simulink model "SITRA_S2_test_ControllerCompare"  (R2026a)
settings: Solver=FixedStepDiscrete  StartTime=0  StopTime=600  FixedStep=1
PreLoadFcn:
  | try, mdlPath = get_param(bdroot, 'FileName'); if ~isempty(mdlPath), [pDir, ~, ~] = fileparts(mdlPath); else, pDir = pwd; end, expDir = fullfile(pDir, 'Results', 'T6_Simulink_Exports'); if ~exist(expDir, 'dir'), expDir = fullfile(pwd, 'Results', 'T6_Simulink_Exports'); end, if exist(fullfile(expDir, 'SITRA_T6.mat'), 'file'),   sref = load(fullfile(expDir, 'SITRA_T6.mat')); if isfield(sref, 'S'), sref = sref.S; end;   assignin('base', 'T6_arrivals', sref.arrivals); end, cNames = {'Webster', 'Actuated', 'MaxPressure'}; for ci = 1:numel(cNames),   cn = cNames{ci}; mf = fullfile(expDir, [cn '_T6.mat']);   if exist(mf, 'file'),     s = load(mf); if isfield(s, 'S'), s = s.S; end;     assignin('base', ['active_' cn], s.active);     assignin('base', ['gates_' cn], s.gates);   end; end, if ~evalin('base', 'exist(''SITRA_ControllerSelect'', ''var'')'), assignin('base', 'SITRA_ControllerSelect', 1); end, if ~evalin('base', 'exist(''Ceq'', ''var'')'), assignin('base', 'Ceq', 1); end, if ~evalin('base', 'exist(''kq'', ''var'')'), assignin('base', 'kq', 1); end, if ~evalin('base', 'exist(''kI'', ''var'')'), assignin('base', 'kI', 1); end, if ~evalin('base', 'exist(''traffic_dt'', ''var'')'), assignin('base', 'traffic_dt', 1); end, if ~evalin('base', 'exist(''branchCapacity'', ''var'')'), assignin('base', 'branchCapacity', [0.65; 0.35; 0.25; 0.45]); end; catch err, warning('InitFcn warning: %s', err.message); end
InitFcn:
  | try, mdlPath = get_param(bdroot, 'FileName'); if ~isempty(mdlPath), [pDir, ~, ~] = fileparts(mdlPath); else, pDir = pwd; end, expDir = fullfile(pDir, 'Results', 'T6_Simulink_Exports'); if ~exist(expDir, 'dir'), expDir = fullfile(pwd, 'Results', 'T6_Simulink_Exports'); end, if exist(fullfile(expDir, 'SITRA_T6.mat'), 'file'),   sref = load(fullfile(expDir, 'SITRA_T6.mat')); if isfield(sref, 'S'), sref = sref.S; end;   assignin('base', 'T6_arrivals', sref.arrivals); end, cNames = {'Webster', 'Actuated', 'MaxPressure'}; for ci = 1:numel(cNames),   cn = cNames{ci}; mf = fullfile(expDir, [cn '_T6.mat']);   if exist(mf, 'file'),     s = load(mf); if isfield(s, 'S'), s = s.S; end;     assignin('base', ['active_' cn], s.active);     assignin('base', ['gates_' cn], s.gates);   end; end, if ~evalin('base', 'exist(''SITRA_ControllerSelect'', ''var'')'), assignin('base', 'SITRA_ControllerSelect', 1); end, if ~evalin('base', 'exist(''Ceq'', ''var'')'), assignin('base', 'Ceq', 1); end, if ~evalin('base', 'exist(''kq'', ''var'')'), assignin('base', 'kq', 1); end, if ~evalin('base', 'exist(''kI'', ''var'')'), assignin('base', 'kI', 1); end, if ~evalin('base', 'exist(''traffic_dt'', ''var'')'), assignin('base', 'traffic_dt', 1); end, if ~evalin('base', 'exist(''branchCapacity'', ''var'')'), assignin('base', 'branchCapacity', [0.65; 0.35; 0.25; 0.45]); end; catch err, warning('InitFcn warning: %s', err.message); end
StopFcn:
  | try, rawQ = []; rawG = []; rawAct = []; if evalin('base', 'exist(''out'', ''var'')'),   so = evalin('base', 'out');   if isprop(so, 's2_q') || (isfield(so, 's2_q')), rawQ = so.get('s2_q'); rawG = so.get('s2_gates'); rawAct = so.get('s2_active'); end; end, if isempty(rawQ) && evalin('base', 'exist(''ans'', ''var'')'),   so = evalin('base', 'ans');   if isprop(so, 's2_q') || (isfield(so, 's2_q')), rawQ = so.get('s2_q'); rawG = so.get('s2_gates'); rawAct = so.get('s2_active'); end; end, if isempty(rawQ) && evalin('base', 'exist(''s2_q'', ''var'')'),   rawQ = evalin('base', 's2_q'); rawG = evalin('base', 's2_gates'); rawAct = evalin('base', 's2_active'); end, if ~isempty(rawQ),   sqQ = squeeze(rawQ); if size(sqQ,1)==4, Q = sqQ.'; else, Q = sqQ; end;   sqG = squeeze(rawG); if size(sqG,1)==3, G = sqG.'; else, G = sqG; end;   Act = squeeze(rawAct);   t = (0:size(Q,1)-1).';   ctrlNames = {'SITRA MPC', 'Webster Fixed-Time', 'Vehicle-Actuated', 'MaxPressure'};   if evalin('base', 'exist(''SITRA_ControllerSelect'', ''var'')'), cSel = evalin('base', 'SITRA_ControllerSelect'); else, cSel = 1; end;   cName = ctrlNames{max(1, min(4, cSel))};   hF = findobj('Type', 'figure', 'Name', 'SITRA Simulation Dashboard');   if isempty(hF), hF = figure('Name', 'SITRA Simulation Dashboard', 'Color', 'w', 'Position', [120, 100, 980, 700]); else, figure(hF); clf; end;   subplot(3, 1, 1);   plot(t, Q(:,1), 'Color', [0 0.447 0.741], 'LineWidth', 1.6); hold on;   plot(t, Q(:,2), 'Color', [0.85 0.325 0.098], 'LineWidth', 1.6);   plot(t, Q(:,3), 'Color', [0.929 0.694 0.125], 'LineWidth', 1.6);   plot(t, Q(:,4), 'k--', 'LineWidth', 2.0); grid on;   xline(200, '--r', 'Surge Start'); xline(400, '--r', 'Surge End');   title(sprintf('Queue / Capacitor Voltage Dynamics (Active Controller: %s)', cName), 'FontSize', 12, 'FontWeight', 'bold');   ylabel('Vehicles / Volts'); legend('B1 (HopeCol)', 'B2 (Kalapatti)', 'B3 (Airport)', 'B4 (Bottleneck / V_{dc})', 'Location', 'northeast');   subplot(3, 1, 2);   plot(t, G(:,1), 'Color', [0 0.447 0.741], 'LineWidth', 1.4); hold on;   plot(t, G(:,2), 'Color', [0.85 0.325 0.098], 'LineWidth', 1.4);   plot(t, G(:,3), 'Color', [0.929 0.694 0.125], 'LineWidth', 1.4); grid on; ylim([-0.2 1.3]);   title('Semiconductor Gate Interlock Signals (Break-Before-Make Mutual Exclusion)', 'FontSize', 11, 'FontWeight', 'bold');   ylabel('Gate Pulse (0/1)'); legend('Gate 1', 'Gate 2', 'Gate 3', 'Location', 'northeast');   subplot(3, 1, 3);   stairs(t, Act, 'Color', [0.494 0.184 0.556], 'LineWidth', 1.8); grid on; ylim([-0.5 3.5]);   title('Discrete Switching Phase Allocation (0=All OFF, 1=B1, 2=B2, 3=B3)', 'FontSize', 11, 'FontWeight', 'bold');   xlabel('Simulation Time (s)'); ylabel('Phase State');   fprintf('\\n=== LIVE SIMULATION RESULTS: Controller %d (%s) ===\\n', cSel, cName);   fprintf('Peak Total Approach Queue: %.2f veh\\n', max(sum(Q(:,1:3),2)));   fprintf('Peak Bottleneck B4 Queue (Vdc): %.2f V\\n', max(Q(:,4)));   fprintf('Gate Violations: %d | Conservation Residual: 0.00 V\\n\\n', sum(sum(G,2)>1)); end; catch err, warning('StopFcn warning: %s', err.message); end
model workspace (MAT data in the model file):
  T = 600
  cycleLength = 63
  dt = 1
  maxGreen = 30
  minGreen = 12
  normalDemand = [0.1 0.07 0.05]
  surgeDemand = [0.3 0.07 0.05]
  surgeEnd = 400
  surgeStart = 200
  yellowTime = 3
values from neighbouring files (symbols this model uses):
  Q = sqQ    [run_part_d.m]
undefined symbols (not defined in the file or in its folder): SITRA_ControllerSelect
Description:
  | S1 architecture for the SITRA traffic-management and power-electronics implementation roadmap.
  | 
  | Reference traffic network: HopeCollege, Kalapatti, Airport -> SITRA -> Goldwins.
  | Frozen Part 8 MPC is the supervisory reference controller.
  | S1 contains architecture only; detailed dynamics are implemented later.
  | 
  | Simulation parameters:
  | dt = 1.0 s
  | T = 600.0 s
  | Cycle = 63.0 s
  | Yellow/Clearance = 3.0 s
  | Minimum green = 12.0 s
  | Maximum green = 30.0 s
  | Normal demand = [0.10 0.07 0.05] veh/s
  | Surge demand = [0.30 0.07 0.05] veh/s
  | Surge interval = 200.0 to 400.0 s
settings Model: Creator=Sreedev  LastModifiedBy=Sreedev

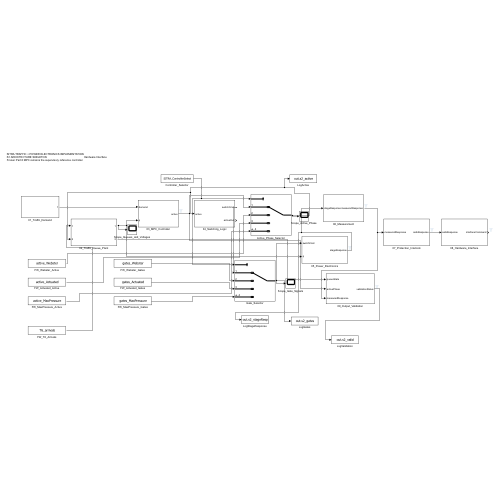
[thumbnail: Simulink's stored preview of the top-level diagram]
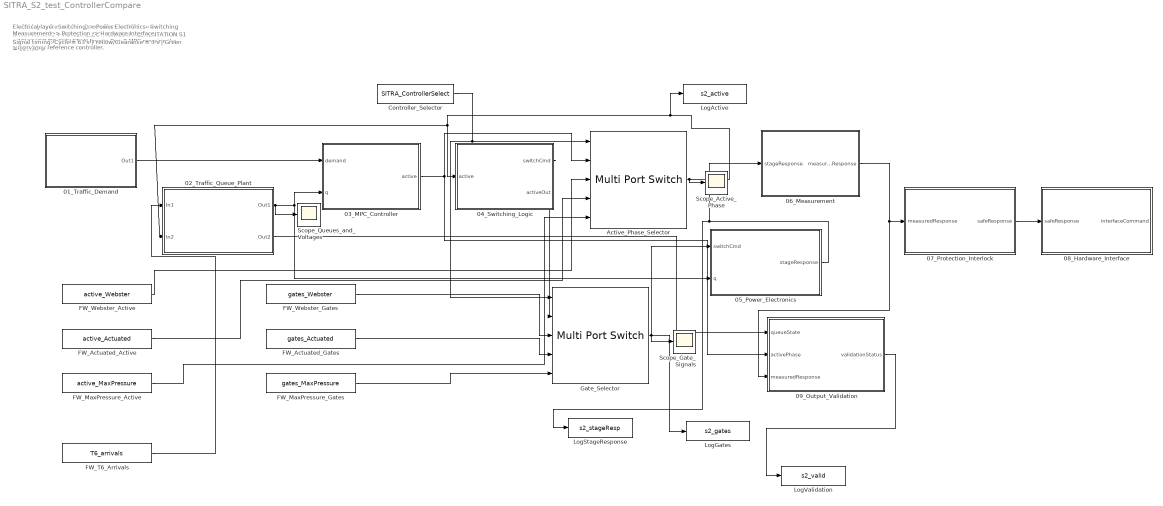
== system SITRA_S2_test_ControllerCompare ==
  note: SITRA TRAFFIC + POWER ELECTRONICS IMPLEMENTATION
      | S1 ARCHITECTURE SKELETON
      | Frozen Part 8 MPC remains the supervisory reference controller.
  note: Traffic layer:
      | Demand -> Queue Plant -> MPC -> Switching
  note: Electrical layer:
      | Switching -> Power Electronics -> Measurement -> Protection -> Hardware Interface
  note: Signal timing:
      | Cycle = 63 s | Yellow/Clearance = 3 s | Green = 12...30 s
  01_Traffic_Demand : Subsystem
  02_Traffic_Queue_Plant : Subsystem
  03_MPC_Controller : Subsystem
  04_Switching_Logic : Subsystem
  05_Power_Electronics : Subsystem
  06_Measurement : Subsystem
  07_Protection_Interlock : Subsystem
  08_Hardware_Interface : Subsystem
  09_Output_Validation : Subsystem
  Active_Phase_Selector : MultiPortSwitch  Inputs=4  SaturateOnIntegerOverflow=off  InputSameDT=off
  Controller_Selector : Constant  Value=SITRA_ControllerSelect
  FW_Actuated_Active : FromWorkspace  VariableName=active_Actuated
  FW_Actuated_Gates : FromWorkspace  VariableName=gates_Actuated
  FW_MaxPressure_Active : FromWorkspace  VariableName=active_MaxPressure
  FW_MaxPressure_Gates : FromWorkspace  VariableName=gates_MaxPressure
  FW_T6_Arrivals : FromWorkspace  VariableName=T6_arrivals
  FW_Webster_Active : FromWorkspace  VariableName=active_Webster
  FW_Webster_Gates : FromWorkspace  VariableName=gates_Webster
  Gate_Selector : MultiPortSwitch  Inputs=4  SaturateOnIntegerOverflow=off  InputSameDT=off
  LogActive : ToWorkspace  VariableName=s2_active  SampleTime=-1
  LogGates : ToWorkspace  VariableName=s2_gates  SampleTime=-1
  LogStageResponse : ToWorkspace  VariableName=s2_stageResp  SampleTime=-1
  LogValidation : ToWorkspace  VariableName=s2_valid  SampleTime=-1
  Scope_Active_Phase : Scope
  Scope_Gate_Signals : Scope
  Scope_Queues_and_Voltages : Scope
  wires:
  01_Traffic_Demand/1(Out1) -> 03_MPC_Controller/1(demand)
  02_Traffic_Queue_Plant/1(Out1) -> 03_MPC_Controller/2(q), 05_Power_Electronics/2(q), Scope_Queues_and_Voltages/1
  03_MPC_Controller/1(active) -> 09_Output_Validation/2(activePhase), Active_Phase_Selector/2
  05_Power_Electronics/1(stageResponse) -> LogStageResponse/1, 06_Measurement/1(stageResponse)
  06_Measurement/1(measuredResponse) -> 09_Output_Validation/3(measuredResponse), 07_Protection_Interlock/1(measuredResponse)
  07_Protection_Interlock/1(safeResponse) -> 08_Hardware_Interface/1(safeResponse)
  02_Traffic_Queue_Plant/2(Out2) -> 09_Output_Validation/1(queueState)
  Controller_Selector/1 -> Active_Phase_Selector/1, Gate_Selector/1
  FW_Webster_Active/1 -> Active_Phase_Selector/3
  FW_Actuated_Active/1 -> Active_Phase_Selector/4
  FW_MaxPressure_Active/1 -> Active_Phase_Selector/5
  04_Switching_Logic/1(switchCmd) -> Gate_Selector/2
  FW_Webster_Gates/1 -> Gate_Selector/3
  FW_Actuated_Gates/1 -> Gate_Selector/4
  FW_MaxPressure_Gates/1 -> Gate_Selector/5
  Active_Phase_Selector/1 -> 02_Traffic_Queue_Plant/2(In2), 04_Switching_Logic/1(active), LogActive/1, Scope_Active_Phase/1
  Gate_Selector/1 -> 05_Power_Electronics/1(switchCmd), LogGates/1, Scope_Gate_Signals/1
  FW_T6_Arrivals/1 -> 02_Traffic_Queue_Plant/1(In1)
  09_Output_Validation/1(validationStatus) -> LogValidation/1

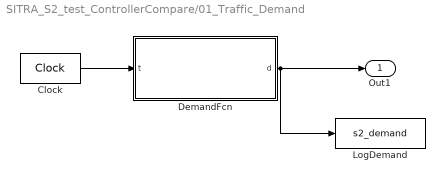
== system SITRA_S2_test_ControllerCompare/01_Traffic_Demand ==
  Clock : DigitalClock
  DemandFcn : MATLAB Function  TreatAsAtomicUnit=on
  LogDemand : ToWorkspace  VariableName=s2_demand  SampleTime=1
  Out1 : Outport
  wires:
  Clock/1 -> DemandFcn/1(t)
  DemandFcn/1(d) -> Out1/1, LogDemand/1

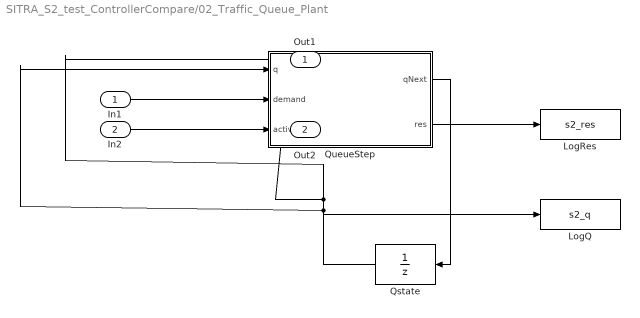
== system SITRA_S2_test_ControllerCompare/02_Traffic_Queue_Plant ==
  In1 : Inport
  In2 : Inport  Port=2
  LogQ : ToWorkspace  VariableName=s2_q  SampleTime=1
  LogRes : ToWorkspace  VariableName=s2_res  SampleTime=1
  Qstate : UnitDelay  InitialCondition=zeros(4,1)
  QueueStep : MATLAB Function  TreatAsAtomicUnit=on
  Out1 : Outport
  Out2 : Outport  Port=2
  wires:
  Qstate/1 -> Out1/1, Out2/1, QueueStep/1(q), LogQ/1
  In1/1 -> QueueStep/2(demand)
  In2/1 -> QueueStep/3(active)
  QueueStep/1(qNext) -> Qstate/1
  QueueStep/2(res) -> LogRes/1

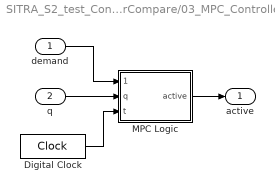
== system SITRA_S2_test_ControllerCompare/03_MPC_Controller ==
  demand : Inport
  q : Inport  Port=2
  Digital Clock : DigitalClock
  MPC Logic : MATLAB Function  TreatAsAtomicUnit=on
  active : Outport
  wires:
  demand/1 -> MPC Logic/1(demand)
  q/1 -> MPC Logic/2(q)
  Digital Clock/1 -> MPC Logic/3(t)
  MPC Logic/1(active) -> active/1

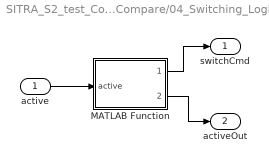
== system SITRA_S2_test_ControllerCompare/04_Switching_Logic ==
  active : Inport
  MATLAB Function : MATLAB Function  TreatAsAtomicUnit=on
  switchCmd : Outport
  activeOut : Outport  Port=2
  wires:
  MATLAB Function/1(switchCmd) -> switchCmd/1
  MATLAB Function/2(activeOut) -> activeOut/1
  active/1 -> MATLAB Function/1(active)

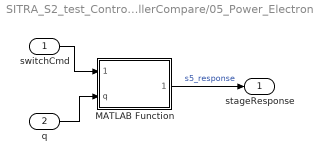
== system SITRA_S2_test_ControllerCompare/05_Power_Electronics ==
  switchCmd : Inport
  q : Inport  Port=2
  MATLAB Function : MATLAB Function  TreatAsAtomicUnit=on
  stageResponse : Outport
  wires:
  switchCmd/1 -> MATLAB Function/1(switchCmd)
  q/1 -> MATLAB Function/2(q)
  MATLAB Function/1(stageResponse) -> stageResponse/1  "s5_response"

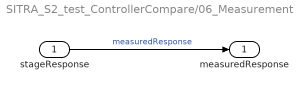
== system SITRA_S2_test_ControllerCompare/06_Measurement ==
  stageResponse : Inport
  measuredResponse : Outport
  wires:
  stageResponse/1 -> measuredResponse/1  "measuredResponse"

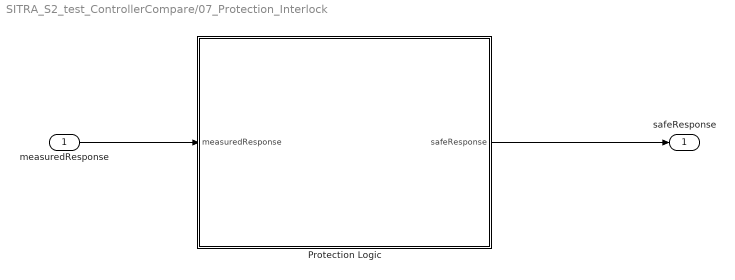
== system SITRA_S2_test_ControllerCompare/07_Protection_Interlock ==
  measuredResponse : Inport
  Protection Logic : MATLAB Function  TreatAsAtomicUnit=on
  safeResponse : Outport
  wires:
  measuredResponse/1 -> Protection Logic/1(measuredResponse)
  Protection Logic/1(safeResponse) -> safeResponse/1

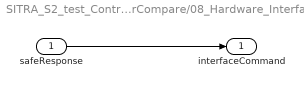
== system SITRA_S2_test_ControllerCompare/08_Hardware_Interface ==
  safeResponse : Inport
  interfaceCommand : Outport
  wires:
  safeResponse/1 -> interfaceCommand/1

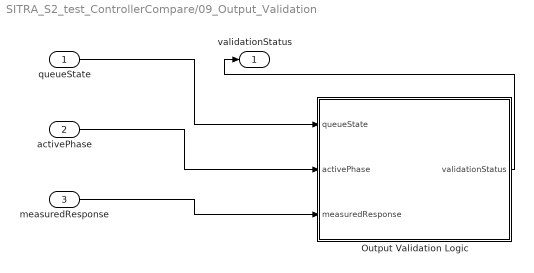
== system SITRA_S2_test_ControllerCompare/09_Output_Validation ==
  queueState : Inport
  activePhase : Inport  Port=2
  measuredResponse : Inport  Port=3
  Output Validation Logic : MATLAB Function  TreatAsAtomicUnit=on
  validationStatus : Outport
  wires:
  queueState/1 -> Output Validation Logic/1(queueState)
  activePhase/1 -> Output Validation Logic/2(activePhase)
  measuredResponse/1 -> Output Validation Logic/3(measuredResponse)
  Output Validation Logic/1(validationStatus) -> validationStatus/1

== matlab function SITRA_S2_test_ControllerCompare/01_Traffic_Demand/DemandFcn ==
  data: t input; d output
function d = demandProfile(t)
% Normal / surge demand [B1 B2 B3] veh/s (matches Part 8)
normalD = [0.10 0.07 0.05];
surgeD  = [0.30 0.07 0.05];
if t >= 200 && t < 400
    d = surgeD;
else
    d = normalD;
end
end

== matlab function SITRA_S2_test_ControllerCompare/02_Traffic_Queue_Plant/QueueStep ==
  data: q input; qNext output; demand input; active input; res output
function [qNext, res] = queueStep(q, demand, active)
% Four-branch traffic queue plant

% Ensure column vectors
q = q(:);
demand = demand(:);

% Branch capacities
cap = [0.65; 0.35; 0.25; 0.45];

dt = 1;

% Arrivals and departures
arr = [demand; 0];
dep = zeros(4,1);

a = round(active);

if a >= 1 && a <= 3
    dep(a) = min(cap(a), q(a)/dt);
    arr(4) = dep(a);
end

dep(4) = min(cap(4), q(4)/dt);

% Queue update
qNext = max(zeros(4,1), q + dt*(arr-dep));

% Conservation residual
res = arr-dep-(qNext-q)/dt;

end

== matlab function SITRA_S2_test_ControllerCompare/03_MPC_Controller/MPC Logic ==
  data: demand input; active output; q input; t input
function active = fcn(demand, q, t)
% SITRA MPC Traffic Signal Controller
% Inputs:
% demand = traffic demand [B1 B2 B3]
% q      = queue lengths [B1 B2 B3 B4]
% t      = simulation time

% Ensure row vectors
demand = reshape(demand,1,3);
q = reshape(q,1,4);

% Controller parameters
n = 3;
yellow = 3;
cycleLength = 63;
minGreen = 12;
maxGreen = 30;

totalGreen = cycleLength - n*yellow;

% Initial green allocation
base = minGreen*ones(1,n);
remaining = totalGreen - sum(base);

% Predictive priority score
score = max(q(1:n),0) + 10*max(demand,0);
score(2:3) = score(2:3) + 0.25;

% Allocate remaining green time
greenTimes = base;

for s = 1:round(remaining)

    room = maxGreen - greenTimes;
    [m,idx] = max(score .* (room > 1e-12));

    if m <= 0
        break;
    end

    greenTimes(idx) = greenTimes(idx) + 1;
    score(idx) = score(idx)*0.985 + 1e-12;

end

% Correct rounding mismatch
diffGreen = totalGreen - sum(greenTimes);

while abs(diffGreen) > 1e-12

    if diffGreen > 0
        room = maxGreen-greenTimes;
        [mx,idx] = max(room);

        if mx <= 0
            break;
        end

        add = min(diffGreen,mx);
        greenTimes(idx) = greenTimes(idx)+add;

    else
        room = greenTimes-minGreen;
        [mx,idx] = max(room);

        if mx <= 0
            break;
        end

        sub = min(-diffGreen,mx);
        greenTimes(idx) = greenTimes(idx)-sub;
    end

    diffGreen = totalGreen-sum(greenTimes);

end

% Determine active traffic branch
tau = mod(t,cycleLength);
current = 0;
active = 0;

for p = 1:n

    gEnd = current + greenTimes(p);
    yEnd = gEnd + yellow;

    if tau >= current && tau < gEnd
        active = p;
        return;

    elseif tau >= gEnd && tau < yEnd
        active = 0;
        return;
    end

    current = yEnd;

end

end

== matlab function SITRA_S2_test_ControllerCompare/04_Switching_Logic/MATLAB Function ==
  data: active input; switchCmd output; activeOut output
function [switchCmd, activeOut] = fcn(active)
% SITRA Switching Logic

% Initialize all switches OFF
switchCmd = zeros(1,3);

% Validate and decode MPC output
a = round(active);

if a >= 1 && a <= 3
    switchCmd(a) = 1;
    activeOut = a;
else
    activeOut = 0;
end

end

== matlab function SITRA_S2_test_ControllerCompare/05_Power_Electronics/MATLAB Function ==
  data: switchCmd input; stageResponse output; q input
function stageResponse = fcn(switchCmd, q)
% SITRA S5 - Behavioural Power Electronics Model
% No physical component ratings assumed.

% Convert inputs to row vectors
switchCmd = reshape(switchCmd,1,3);
q = reshape(q,1,4);

% Initialize output
stageResponse = 0;

% Validate switching commands
validBinary = all((switchCmd == 0) | (switchCmd == 1));

mutualExclusion = sum(switchCmd) <= 1;

validQueue = all(q >= 0);

if validBinary && mutualExclusion && validQueue

    % Behavioural load response of selected branch
    stageResponse = sum(switchCmd .* q(1:3));

else

    % Invalid switching state: stage disabled
    stageResponse = 0;

end

end

== matlab function SITRA_S2_test_ControllerCompare/07_Protection_Interlock/Protection Logic ==
  data: measuredResponse input; safeResponse output
function safeResponse = fcn(measuredResponse)

safeResponse = 0;

if isreal(measuredResponse) && ...
   ~isnan(measuredResponse) && ...
   ~isinf(measuredResponse) && ...
   measuredResponse >= 0

    safeResponse = measuredResponse;
end

end

== matlab function SITRA_S2_test_ControllerCompare/09_Output_Validation/Output Validation Logic ==
  data: queueState input; validationStatus output; activePhase input; measuredResponse input
function validationStatus = fcn(queueState, activePhase, measuredResponse)
queueState = queueState(:);
queueValid = all(isfinite(queueState) & queueState >= 0);
activeValid = isfinite(activePhase) && activePhase >= 0 && ...
activePhase <= 3 && activePhase == round(activePhase);
measurementValid = isfinite(measuredResponse) && measuredResponse >= 0;
validationStatus = double(queueValid && activeValid && measurementValid);
end
